simulink model "MiL"  (R2026a)
settings: Solver=FixedStepAuto  StartTime=0  StopTime=2  FixedStep=1e-3  MaxStep=1e-3  EnableMultiTasking=on
values from neighbouring files (symbols this model uses):
  effective_bulkmodulus = 750e6    (= 750000000)    [parameters.m]
  m_load = 58    [parameters.m]
  p_supply = 90e5    (= 9000000)    [parameters.m]
  p_tank = 1.01325e5    (= 101325)    [parameters.m]
undefined symbols (not defined in the file or in its folder): cyl, pipe, valve
libraries: slpidlib x1
settings Model: Creator=ranta34  LastModifiedBy=Lenovo Yoga
settings DataIOCC: SignalLoggingSaveFormat=ModelDataLogs  TimeSaveName=t_sim  Refine=3
settings OptimizationCC: InitFltsAndDblsToZero=on
settings DebuggingCC: SaveWithParameterizedLinksMsg=none  UnderspecifiedInitializationDetection=Classic  SignalResolutionControl=TryResolveAllWithWarning  MinStepSizeMsg=error  MultiTaskDSMMsg=warning  MultiTaskCondExecSysMsg=none
settings HardwareCC: ProdHWDeviceType=32-bit Generic
settings GRTTargetCC: TargetFcnLib=ansi_tfl_tmw.mat  CombineOutputUpdateFcns=off  GRTInterface=on

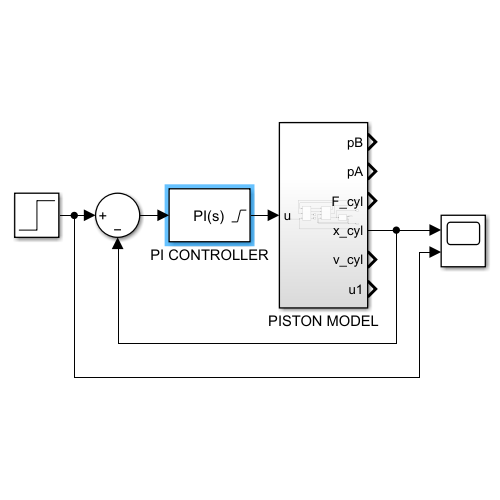
[thumbnail: Simulink's stored preview of the top-level diagram]
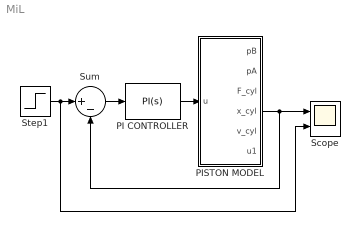
== system MiL ==
  PI CONTROLLER : slpidlib/PID Controller  Controller=PI  Form=Parallel  TimeDomain=Continuous-time  UseExternalTs=off  SampleTime=-1  IntegratorMethod=Forward Euler  FilterMethod=Forward Euler  ControllerParametersSource=internal  P=60  I=1  UseKiTs=off  D=0  UseExternalDerivativeSource=off  N=100  UseFilter=on  TunerSelectOption=Transfer Function Based (PID Tuner App)  InitialConditionSource=internal  InitialConditionForIntegrator=0  InitialConditionForFilter=0  DifferentiatorICPrevScaledInput=0  ExternalReset=none  TrackingMode=off  Kt=1  LimitOutput=on  SatLimitsSource=internal  UpperSaturationLimit=1  LowerSaturationLimit=-1  LinearizeAsGain=on  AntiWindupMode=clamping  Kb=1  LimitIntegrator=off  UpperIntegratorSaturationLimit=inf  LowerIntegratorSaturationLimit=-inf  POutMin=[]  POutMax=[]  IOutMin=[]  IOutMax=[]  DOutMin=[]  DOutMax=[]  NOutMin=[]  NOutMax=[]  SumOutMin=[]  SumOutMax=[]  SaturationOutMin=[]  SaturationOutMax=[]  PParamMin=[]  PParamMax=[]  IParamMin=[]  IParamMax=[]  DParamMin=[]  DParamMax=[]  NParamMin=[]  NParamMax=[]  KbParamMin=[]  KbParamMax=[]  KtParamMin=[]  KtParamMax=[]  KbOutMin=[]  KbOutMax=[]  KtOutMin=[]  KtOutMax=[]  IntegratorOutMin=[]  IntegratorOutMax=[]  FilterOutMin=[]  FilterOutMax=[]  SumI1OutMin=[]  SumI1OutMax=[]  SumI2OutMin=[]  SumI2OutMax=[]  SumI3OutMin=[]  SumI3OutMax=[]  SumI4OutMin=[]  SumI4OutMax=[]  SumDOutMin=[]  SumDOutMax=[]  DifferentiatorOutMin=[]  DifferentiatorOutMax=[]  FilterDiffOutCoefMin=[]  FilterDiffOutCoefMax=[]  ReciprocalOutMin=[]  ReciprocalOutMax=[]  SumDenOutMin=[]  SumDenOutMax=[]  SumNumOutMin=[]  SumNumOutMax=[]  DivideOutMin=[]  DivideOutMax=[]  UdiffTsProdOutMin=[]  UdiffTsProdOutMax=[]  NTsProdOutMin=[]  NTsProdOutMax=[]  UintegralTsProdOutMin=[]  UintegralTsProdOutMax=[]  UngainTsProdOutMin=[]  UngainTsProdOutMax=[]  ClampingZeroOutDataTypeStr=Inherit: Inherit via back propagation  ClampingZeroOutMin=[]  ClampingZeroOutMax=[]  FilterDenConstantOutDataTypeStr=Inherit: Inherit via back propagation  FilterDenConstantOutMin=[]  FilterDenConstantOutMax=[]  PCopyOutDataTypeStr=Inherit: Inherit via back propagation  PCopyOutMin=[]  PCopyOutMax=[]  NCopyOutDataTypeStr=Inherit: Inherit via back propagation  NCopyOutMin=[]  NCopyOutMax=[]  IntegratorContinuousStateAttributes=''  IntegratorStateMustResolveToSignalObject=off  IntegratorRTWStateStorageClass=Auto  FilterContinuousStateAttributes=''  FilterStateMustResolveToSignalObject=off  FilterRTWStateStorageClass=Auto  ParallelPVariant=InternalParameters  IdealPVariant=Disabled  IVariant=InternalParameters  DVariant=Disabled  IntegratorVariant=Continuous  SatVariant=Enabled  AWVariant=ContClampingParallel  PCopyVariant=Disabled  TRVariant=Disabled  FdbkBlocksVariant=Forward  IdealPFdbkVariant=Disabled  SatFdbkVariant=Disabled  DerivativeFilterVariant=Disabled  NVariant=Disabled  NCopyVariant=Disabled_SignalSpec  FilterICVariant=Disabled  IntegratorICVariant=InternalICs  ExternalResetVariant=Disabled  TRSumVariant=Passthrough  SumFdbkVariant=Disabled  SumVariant=Sum_PI  TsampFilterVariant=InternalTs  TsampNgainVariant=Passthrough  TsampIntegralVariant=Disabled_SignalSpec  ExternalSaturationOutDataTypeStr=Inherit: Same as second input  DerivativeSourceVariant=Disabled  PreIntVariant=InternalPreInt
  PISTON MODEL : Subsystem
  Scope : Scope  NumInputPorts=2
      settings: ActiveDisplayYMinimum=-0.44593920723278446  ActiveDisplayYMaximum=1.0292768833436203
  Step1 : Step  Time=0.5  FinalValue=0.40  SampleTime=0
  Sum : Sum  Inputs=|+-
  wires:
  Sum/1 -> PI CONTROLLER/1
  Step1/1 -> Scope/2, Sum/1
  PISTON MODEL/4(x_cyl) -> Scope/1, Sum/2
  PI CONTROLLER/1 -> PISTON MODEL/1(u)

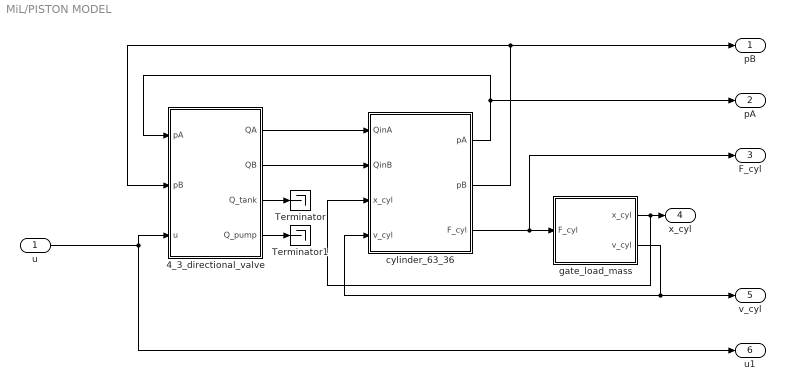
== system MiL/PISTON MODEL ==
  u : Inport
  4_3_directional_valve : Subsystem
  Terminator : Terminator
  Terminator1 : Terminator
  cylinder_63_36 : Subsystem
  gate_load_mass : Subsystem
  pB : Outport
  pA : Outport  Port=2
  F_cyl : Outport  Port=3
  x_cyl : Outport  Port=4
  v_cyl : Outport  Port=5
  u1 : Outport  Port=6
  wires:
  u/1 -> u1/1, 4_3_directional_valve/3(u)
  cylinder_63_36/1(pA) -> pA/1, 4_3_directional_valve/1(pA)
  cylinder_63_36/2(pB) -> pB/1, 4_3_directional_valve/2(pB)
  4_3_directional_valve/1(QA) -> cylinder_63_36/1(QinA)
  4_3_directional_valve/2(QB) -> cylinder_63_36/2(QinB)
  4_3_directional_valve/4(Q_pump) -> Terminator1/1
  4_3_directional_valve/3("Q_tank ") -> Terminator/1
  cylinder_63_36/3(F_cyl) -> F_cyl/1, gate_load_mass/1(F_cyl)
  gate_load_mass/2(v_cyl) -> v_cyl/1, cylinder_63_36/4(v_cyl)
  gate_load_mass/1(x_cyl) -> cylinder_63_36/3(x_cyl), x_cyl/1

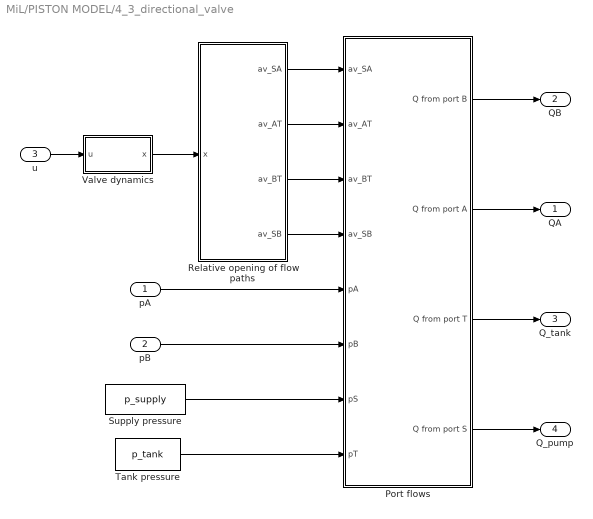
== system MiL/PISTON MODEL/4_3_directional_valve ==
  pA : Inport
  pB : Inport  Port=2
  u : Inport  Port=3
  Port flows : Subsystem
  Relative opening of flow paths : Subsystem
  Supply pressure : Constant  Value=p_supply
  Tank pressure : Constant  Value=p_tank
  Valve dynamics : Subsystem
  QA : Outport  VectorParamsAs1DForOutWhenUnconnected=off
  QB : Outport  Port=2  VectorParamsAs1DForOutWhenUnconnected=off
  "Q_tank " : Outport  Port=3  VectorParamsAs1DForOutWhenUnconnected=off
  Q_pump : Outport  Port=4  VectorParamsAs1DForOutWhenUnconnected=off
  wires:
  pA/1 -> Port flows/5(pA)
  pB/1 -> Port flows/6(pB)
  Valve dynamics/1(x) -> Relative opening of flow paths/1(x)
  Port flows/3(Q from port T) -> "Q_tank "/1
  Port flows/4(Q from port S) -> Q_pump/1
  Relative opening of flow paths/1(av_SA) -> Port flows/1(av_SA)
  Relative opening of flow paths/2(av_AT) -> Port flows/2(av_AT)
  Relative opening of flow paths/4(av_SB) -> Port flows/4(av_SB)
  u/1 -> Valve dynamics/1(u)
  Port flows/2(Q from port A) -> QA/1
  Port flows/1(Q from port B) -> QB/1
  Supply pressure/1 -> Port flows/7(pS)
  Tank pressure/1 -> Port flows/8(pT)
  Relative opening of flow paths/3(av_BT) -> Port flows/3(av_BT)

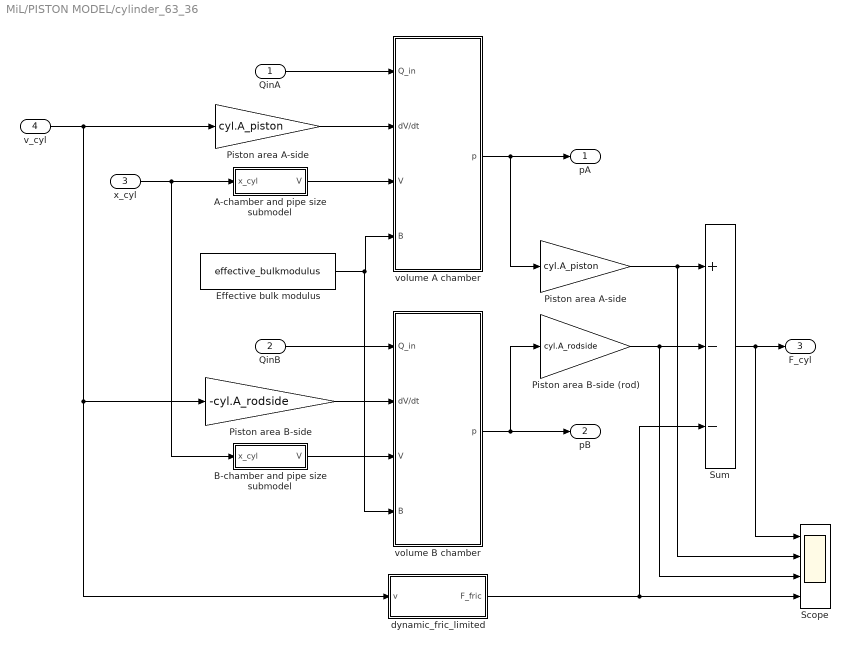
== system MiL/PISTON MODEL/cylinder_63_36 ==
  QinA : Inport
  QinB : Inport  Port=2
  x_cyl : Inport  Port=3
  v_cyl : Inport  Port=4
  A-chamber and pipe size submodel : Subsystem
  B-chamber and pipe size submodel : Subsystem
  Effective bulk modulus : Constant  Value=effective_bulkmodulus
  Piston area A-side : Gain  Gain=cyl.A_piston
  Piston area B-side (rod) : Gain  Gain=cyl.A_rodside
  Piston area A-side : Gain  Gain=cyl.A_piston
  Piston area B-side : Gain  Gain=-cyl.A_rodside
  Scope : Scope  NumInputPorts=4
      settings: ActiveDisplayYMinimum=-3356.48237  ActiveDisplayYMaximum=15799.75819
  Sum : Sum  Inputs=+--
  dynamic_fric_limited : Subsystem
  volume A chamber : Subsystem
  volume B chamber : Subsystem
  pA : Outport  VectorParamsAs1DForOutWhenUnconnected=off
  pB : Outport  Port=2  VectorParamsAs1DForOutWhenUnconnected=off
  F_cyl : Outport  Port=3  VectorParamsAs1DForOutWhenUnconnected=off
  wires:
  Piston area A-side/1 -> Scope/2, Sum/1
  volume A chamber/1(p) -> pA/1, Piston area A-side/1
  x_cyl/1 -> B-chamber and pipe size submodel/1(x_cyl), A-chamber and pipe size submodel/1(x_cyl)
  v_cyl/1 -> dynamic_fric_limited/1(v), Piston area B-side/1, Piston area A-side/1
  Piston area A-side/1 -> volume A chamber/2(" dV/dt")
  Effective bulk modulus/1 -> volume B chamber/4(" B"), volume A chamber/4(" B")
  Sum/1 -> Scope/1, F_cyl/1
  QinA/1 -> volume A chamber/1(Q_in)
  volume B chamber/1(p) -> pB/1, Piston area B-side (rod)/1
  Piston area B-side (rod)/1 -> Scope/3, Sum/2
  A-chamber and pipe size submodel/1(V) -> volume A chamber/3(" V")
  QinB/1 -> volume B chamber/1(Q_in)
  B-chamber and pipe size submodel/1(V) -> volume B chamber/3(" V")
  Piston area B-side/1 -> volume B chamber/2(" dV/dt")
  dynamic_fric_limited/1(F_fric) -> Sum/3, Scope/4

== system MiL/PISTON MODEL/gate_load_mass ==
  F_cyl : Inport
  Add : Sum
  Gain : Gain  Gain=1/m_load
  Integrator : Integrator
  Integrator1 : Integrator  InitialCondition=cyl.x_init
  load_fric : Subsystem
  x_cyl : Outport  VectorParamsAs1DForOutWhenUnconnected=off
  v_cyl : Outport  Port=2  VectorParamsAs1DForOutWhenUnconnected=off
  wires:
  Add/1 -> Gain/1
  Gain/1 -> Integrator/1  "accel"
  Integrator/1 -> load_fric/1(v), v_cyl/1, Integrator1/1  "velocity"
  Integrator1/1 -> x_cyl/1  "position"
  F_cyl/1 -> Add/1
  load_fric/1(F_fric_load) -> Add/2

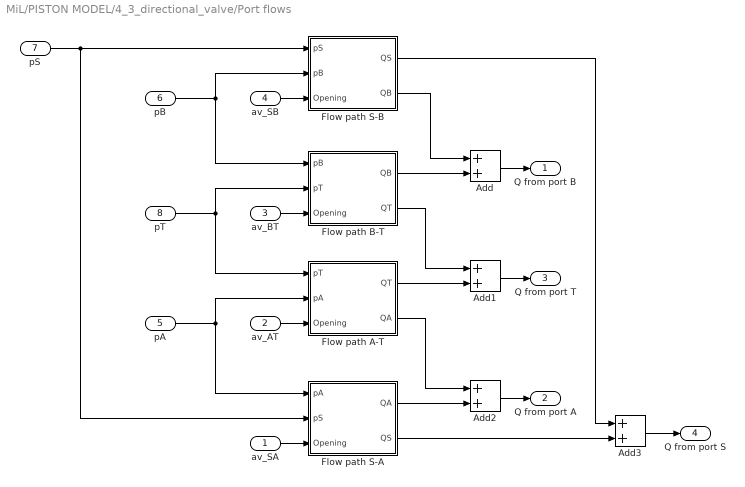
== system MiL/PISTON MODEL/4_3_directional_valve/Port flows ==
  av_SA : Inport
  av_AT : Inport  Port=2
  av_BT : Inport  Port=3
  av_SB : Inport  Port=4
  pA : Inport  Port=5
  pB : Inport  Port=6
  pS : Inport  Port=7
  pT : Inport  Port=8
  Add{,1..3} (4 alike) : Sum
  Flow path A-T : Subsystem  mask(Hydraulic){DPN=valve.dpN, QN=valve.QN, ptr=valve.ptr}
      mask prompts: DPN "Nominal Pressure Difference [Pa] :"; QN "Flow at nominal pressure difference and maximum opening [m^3/s] :"; ptr "Transition pressure [Pa] :"
      mask help:
      | Implements numerically robust turbulent flow equation. Polynomial flow equation is
      | used when abs(dp) is smaller than transition pressure.
      | [Source: Ellman, A. & Piche, R. 1996.
      | A Modified Orifice Flow Formula for Numerical Simulation of Fluid Power Systems.
      | Fluid Power Systems and Technology, ASME]
      mask init:
      | K = QN/(sqrt(DPN));
  Flow path B-T : Subsystem  mask(Hydraulic){DPN=valve.dpN, QN=valve.QN, ptr=valve.ptr}
      mask prompts: DPN "Nominal Pressure Difference [Pa] :"; QN "Flow at nominal pressure difference and maximum opening [m^3/s] :"; ptr "Transition pressure [Pa] :"
      mask help:
      | Implements numerically robust turbulent flow equation. Polynomial flow equation is
      | used when abs(dp) is smaller than transition pressure.
      | [Source: Ellman, A. & Piche, R. 1996.
      | A Modified Orifice Flow Formula for Numerical Simulation of Fluid Power Systems.
      | Fluid Power Systems and Technology, ASME]
      mask init:
      | K = QN/(sqrt(DPN));
  Flow path S-A : Subsystem  mask(Hydraulic){DPN=valve.dpN, QN=valve.QN, ptr=valve.ptr}
      mask prompts: DPN "Nominal Pressure Difference [Pa] :"; QN "Flow at nominal pressure difference and maximum opening [m^3/s] :"; ptr "Transition pressure [Pa] :"
      mask help:
      | Implements numerically robust turbulent flow equation. Polynomial flow equation is
      | used when abs(dp) is smaller than transition pressure.
      | [Source: Ellman, A. & Piche, R. 1996.
      | A Modified Orifice Flow Formula for Numerical Simulation of Fluid Power Systems.
      | Fluid Power Systems and Technology, ASME]
      mask init:
      | K = QN/(sqrt(DPN));
  Flow path S-B : Subsystem  mask(Hydraulic){DPN=valve.dpN, QN=valve.QN, ptr=valve.ptr}
      mask prompts: DPN "Nominal Pressure Difference [Pa] :"; QN "Flow at nominal pressure difference and maximum opening [m^3/s] :"; ptr "Transition pressure [Pa] :"
      mask help:
      | Implements numerically robust turbulent flow equation. Polynomial flow equation is
      | used when abs(dp) is smaller than transition pressure.
      | [Source: Ellman, A. & Piche, R. 1996.
      | A Modified Orifice Flow Formula for Numerical Simulation of Fluid Power Systems.
      | Fluid Power Systems and Technology, ASME]
      mask init:
      | K = QN/(sqrt(DPN));
  Q from port B : Outport  VectorParamsAs1DForOutWhenUnconnected=off
  Q from port A : Outport  Port=2  VectorParamsAs1DForOutWhenUnconnected=off
  Q from port T : Outport  Port=3  VectorParamsAs1DForOutWhenUnconnected=off
  Q from port S : Outport  Port=4  VectorParamsAs1DForOutWhenUnconnected=off
  wires:
  av_SA/1 -> Flow path S-A/3(Opening)
  av_AT/1 -> Flow path A-T/3(Opening)
  av_BT/1 -> Flow path B-T/3(Opening)
  pA/1 -> Flow path A-T/2(pA), Flow path S-A/1(pA)
  pB/1 -> Flow path B-T/1(pB), Flow path S-B/2(pB)
  pS/1 -> Flow path S-B/1(pS), Flow path S-A/2(pS)
  pT/1 -> Flow path A-T/1(pT), Flow path B-T/2(pT)
  Add/1 -> Q from port B/1
  Add1/1 -> Q from port T/1
  Add2/1 -> Q from port A/1
  Add3/1 -> Q from port S/1
  Flow path S-B/1(QS) -> Add3/1
  Flow path S-A/2(QS) -> Add3/2
  Flow path S-A/1(QA) -> Add2/2
  Flow path A-T/2(QA) -> Add2/1
  Flow path A-T/1(QT) -> Add1/2
  Flow path B-T/2(QT) -> Add1/1
  Flow path B-T/1(QB) -> Add/2
  Flow path S-B/2(QB) -> Add/1
  av_SB/1 -> Flow path S-B/3(Opening)

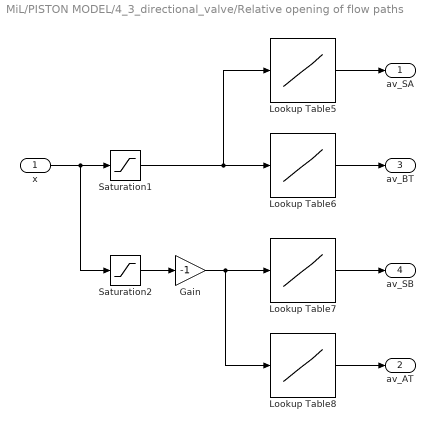
== system MiL/PISTON MODEL/4_3_directional_valve/Relative opening of flow paths ==
  x : Inport
  Gain : Gain  Gain=-1
  Lookup Table5 : Lookup  InputValues=[0.01 0.05 0.1 0.2 0.3 0.4 1]  Table=[0.01 0.039 0.078 0.16 0.23 0.31 0.78]  SaturateOnIntegerOverflow=off
  Lookup Table6 : Lookup  InputValues=[0.01 0.05 0.1 0.2 0.3 0.4 1]  Table=[0.01 0.036 0.072 0.14 0.22 0.29 0.72]  SaturateOnIntegerOverflow=off
  Lookup Table7 : Lookup  InputValues=[0.01 0.05 0.1 0.2 0.3 0.4 1]  Table=[0.01 0.039 0.077 0.15 0.23 0.31 0.77]  SaturateOnIntegerOverflow=off
  Lookup Table8 : Lookup  InputValues=[0.01 0.05 0.1 0.2 0.3 0.4 1]  Table=[0.01 0.035 0.070 0.14 0.21 0.28 0.70]  SaturateOnIntegerOverflow=off
  Saturation1 : Saturate  UpperLimit=1  LowerLimit=0
  Saturation2 : Saturate  UpperLimit=0  LowerLimit=-1
  av_SA : Outport  VectorParamsAs1DForOutWhenUnconnected=off
  av_AT : Outport  Port=2  VectorParamsAs1DForOutWhenUnconnected=off
  av_BT : Outport  Port=3  VectorParamsAs1DForOutWhenUnconnected=off
  av_SB : Outport  Port=4  VectorParamsAs1DForOutWhenUnconnected=off
  wires:
  x/1 -> Saturation2/1, Saturation1/1
  Saturation2/1 -> Gain/1
  Lookup Table8/1 -> av_AT/1
  Lookup Table7/1 -> av_SB/1
  Lookup Table6/1 -> av_BT/1
  Lookup Table5/1 -> av_SA/1
  Saturation1/1 -> Lookup Table5/1, Lookup Table6/1
  Gain/1 -> Lookup Table8/1, Lookup Table7/1

== system MiL/PISTON MODEL/4_3_directional_valve/Valve dynamics ==
  u : Inport
  Rate Limiter : RateLimiter  RisingSlewLimit=valve.ratelimit  FallingSlewLimit=-valve.ratelimit  SampleTimeMode=inherited
  Saturation limits [-1,1] : Saturate  UpperLimit=1  LowerLimit=-1
  Saturation limits [-1,1]2 : Saturate  UpperLimit=1  LowerLimit=-1
  Transfer Fcn1 : TransferFcn  Denominator=[valve.tau 1]
  Transport Delay of the valve : TransportDelay  DelayTime=valve.delay
  x : Outport  VectorParamsAs1DForOutWhenUnconnected=off
  wires:
  Saturation limits [-1,1]/1 -> Transport Delay of the valve/1
  Transport Delay of the valve/1 -> Rate Limiter/1
  Rate Limiter/1 -> Transfer Fcn1/1
  u/1 -> Saturation limits [-1,1]/1
  Transfer Fcn1/1 -> Saturation limits [-1,1]2/1
  Saturation limits [-1,1]2/1 -> x/1

== system MiL/PISTON MODEL/cylinder_63_36/A-chamber and pipe size submodel ==
  x_cyl : Inport
  A : Gain  Gain=pipe.area
  A chamber dead volume : Constant  Value=cyl.V0A
  Add : Sum  Inputs=+++
  Gain : Gain  Gain=cyl.A_piston
  Lenght : Constant  Value=pipe.lenght
  V : Outport  VectorParamsAs1DForOutWhenUnconnected=off
  wires:
  A/1 -> Add/3
  Lenght/1 -> A/1
  A chamber dead volume/1 -> Add/2
  Gain/1 -> Add/1
  x_cyl/1 -> Gain/1
  Add/1 -> V/1

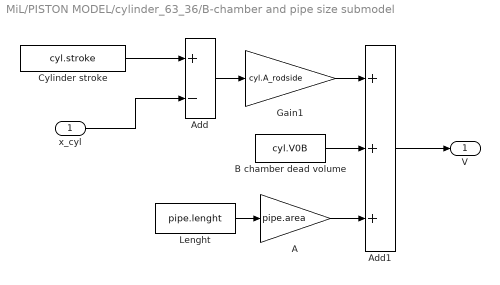
== system MiL/PISTON MODEL/cylinder_63_36/B-chamber and pipe size submodel ==
  x_cyl : Inport
  A : Gain  Gain=pipe.area
  Add : Sum  Inputs=+-
  Add1 : Sum  Inputs=+++
  B chamber dead volume : Constant  Value=cyl.V0B
  Cylinder stroke : Constant  Value=cyl.stroke
  Gain1 : Gain  Gain=cyl.A_rodside
  Lenght : Constant  Value=pipe.lenght
  V : Outport  VectorParamsAs1DForOutWhenUnconnected=off
  wires:
  A/1 -> Add1/3
  Lenght/1 -> A/1
  Cylinder stroke/1 -> Add/1
  Gain1/1 -> Add1/1
  Add/1 -> Gain1/1
  x_cyl/1 -> Add/2
  B chamber dead volume/1 -> Add1/2
  Add1/1 -> V/1

== system MiL/PISTON MODEL/cylinder_63_36/dynamic_fric_limited ==
  v : Inport
  Abs : Abs  SaturateOnIntegerOverflow=off
  Product : Product
  Sign : Signum
  cyl_fric_up_to_100mm/s : Lookup_n-D  NumberOfTableDimensions=1  BreakpointsForDimension1=|  Table=|  InternalRulePriority=Speed  RndMeth=Simplest
      BreakpointsForDimension1=|
      | [0
      | 5
      | 10
      | 15
      | 20
      | 25
      | 30
      | 35
      | 40
      | 45
      | 50
      | 55
      | 60
      | 65
      | 70
      | 75
      | 80
      | 85
      | 90
      | 95
      | 100]./1e3;
      Table=|
      | [0
      | 242
      | 550
      | 838
      | 996
      | 972
      | 850
      | 757
      | 728
      | 733
      | 744
      | 753
      | 759
      | 765
      | 770
      | 775
      | 780
      | 785
      | 790
      | 795
      | 800];
  F_fric : Outport  VectorParamsAs1DForOutWhenUnconnected=off
  wires:
  Abs/1 -> cyl_fric_up_to_100mm/s/1
  v/1 -> Sign/1, Abs/1
  cyl_fric_up_to_100mm/s/1 -> Product/1
  Sign/1 -> Product/2
  Product/1 -> F_fric/1

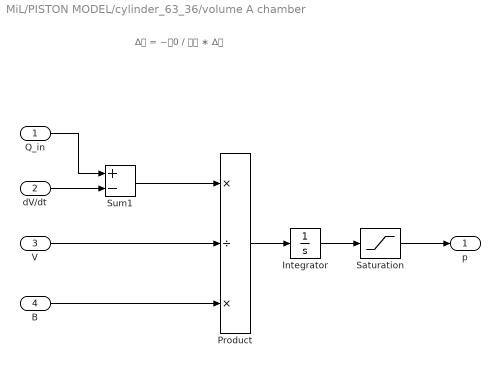
== system MiL/PISTON MODEL/cylinder_63_36/volume A chamber ==
  note: ∆𝑉 = −𝑉0 / 𝐵𝑛 ∗ ∆𝑝
  Q_in : Inport
  " dV/dt" : Inport  Port=2
  " V" : Inport  Port=3
  " B" : Inport  Port=4
  Integrator : Integrator  InitialCondition=cyl.p0A  AbsoluteTolerance=10
  Product : Product  Inputs=*/*  InputSameDT=on  SaturateOnIntegerOverflow=on  OutDataTypeStr=Inherit: Same as first input
  Saturation : Saturate  UpperLimit=inf  LowerLimit=-1e5
  Sum1 : Sum  Inputs=+-  InputSameDT=on  SaturateOnIntegerOverflow=on  OutDataTypeStr=Inherit: Same as first input
  p : Outport  VectorParamsAs1DForOutWhenUnconnected=off
  wires:
  Integrator/1 -> Saturation/1
  Product/1 -> Integrator/1
  Sum1/1 -> Product/1
  " B"/1 -> Product/3
  Saturation/1 -> p/1
  Q_in/1 -> Sum1/1
  " V"/1 -> Product/2
  " dV/dt"/1 -> Sum1/2

== system MiL/PISTON MODEL/cylinder_63_36/volume B chamber ==
  Q_in : Inport
  " dV/dt" : Inport  Port=2
  " V" : Inport  Port=3
  " B" : Inport  Port=4
  Integrator : Integrator  InitialCondition=cyl.p0B  AbsoluteTolerance=10
  Product : Product  Inputs=*/*  InputSameDT=on  SaturateOnIntegerOverflow=on  OutDataTypeStr=Inherit: Same as first input
  Saturation : Saturate  UpperLimit=inf  LowerLimit=-1e5
  Sum1 : Sum  Inputs=+-  InputSameDT=on  SaturateOnIntegerOverflow=on  OutDataTypeStr=Inherit: Same as first input
  p : Outport  VectorParamsAs1DForOutWhenUnconnected=off
  wires:
  " dV/dt"/1 -> Sum1/2
  " V"/1 -> Product/2
  Q_in/1 -> Sum1/1
  Saturation/1 -> p/1
  " B"/1 -> Product/3
  Sum1/1 -> Product/1
  Product/1 -> Integrator/1
  Integrator/1 -> Saturation/1

== system MiL/PISTON MODEL/gate_load_mass/load_fric ==
  v : Inport
  Gain1 : Gain  Gain=-1
  Product : Product  Inputs=4
  Sign : Signum
  coeff_fric : Constant  Value=0.7e5
  F_fric_load : Outport  VectorParamsAs1DForOutWhenUnconnected=off
  wires:
  Product/1 -> F_fric_load/1
  Sign/1 -> Gain1/1
  coeff_fric/1 -> Product/4
  Gain1/1 -> Product/1
  v/1 -> Product/2, Product/3, Sign/1

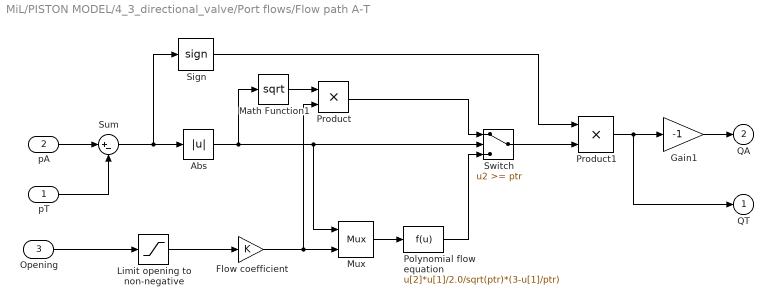
== system MiL/PISTON MODEL/4_3_directional_valve/Port flows/Flow path A-T ==
  pT : Inport
  pA : Inport  Port=2
  Opening : Inport  Port=3
  Abs : Abs  ZeroCross=off
  Flow coefficient : Gain  Gain=K  SaturateOnIntegerOverflow=on  OutDataTypeStr=Inherit: Same as input  ParamDataTypeStr=Inherit: Same as input
  Gain1 : Gain  Gain=-1  SaturateOnIntegerOverflow=on  OutDataTypeStr=Inherit: Same as input  ParamDataTypeStr=Inherit: Same as input
  Limit opening to non-negative : Saturate  UpperLimit=inf  LowerLimit=0
  Math Function1 : Math  Operator=sqrt  SignedPower=on
  Mux : Mux  Inputs=2
  Polynomial flow equation : Fcn  Expr=u[2]*u[1]/2.0/sqrt(ptr)*(3-u[1]/ptr)
  Product : Product  InputSameDT=on  SaturateOnIntegerOverflow=on  OutDataTypeStr=Inherit: Same as first input
  Product1 : Product  InputSameDT=on  SaturateOnIntegerOverflow=on  OutDataTypeStr=Inherit: Same as first input
  Sign : Signum  ZeroCross=off
  Sum : Sum  Inputs=|+-
  Switch : Switch  Threshold=ptr  ZeroCross=off
  QT : Outport  InitialOutput=0  VectorParamsAs1DForOutWhenUnconnected=off
  QA : Outport  Port=2  InitialOutput=0  VectorParamsAs1DForOutWhenUnconnected=off
  wires:
  Opening/1 -> Limit opening to non-negative/1
  Sum/1 -> Abs/1, Sign/1
  Polynomial flow equation/1 -> Switch/3
  Mux/1 -> Polynomial flow equation/1
  Product/1 -> Switch/1
  Math Function1/1 -> Product/1
  Abs/1 -> Mux/1, Switch/2, Math Function1/1
  Limit opening to non-negative/1 -> Flow coefficient/1
  Flow coefficient/1 -> Product/2, Mux/2
  Sign/1 -> Product1/1
  Product1/1 -> Gain1/1, QT/1
  Switch/1 -> Product1/2
  pA/1 -> Sum/1
  pT/1 -> Sum/2
  Gain1/1 -> QA/1

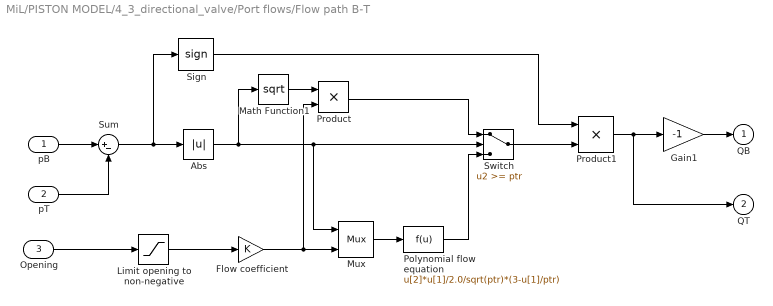
== system MiL/PISTON MODEL/4_3_directional_valve/Port flows/Flow path B-T ==
  pB : Inport
  pT : Inport  Port=2
  Opening : Inport  Port=3
  Abs : Abs  ZeroCross=off
  Flow coefficient : Gain  Gain=K  SaturateOnIntegerOverflow=on  OutDataTypeStr=Inherit: Same as input  ParamDataTypeStr=Inherit: Same as input
  Gain1 : Gain  Gain=-1  SaturateOnIntegerOverflow=on  OutDataTypeStr=Inherit: Same as input  ParamDataTypeStr=Inherit: Same as input
  Limit opening to non-negative : Saturate  UpperLimit=inf  LowerLimit=0
  Math Function1 : Math  Operator=sqrt  SignedPower=on
  Mux : Mux  Inputs=2
  Polynomial flow equation : Fcn  Expr=u[2]*u[1]/2.0/sqrt(ptr)*(3-u[1]/ptr)
  Product : Product  InputSameDT=on  SaturateOnIntegerOverflow=on  OutDataTypeStr=Inherit: Same as first input
  Product1 : Product  InputSameDT=on  SaturateOnIntegerOverflow=on  OutDataTypeStr=Inherit: Same as first input
  Sign : Signum  ZeroCross=off
  Sum : Sum  Inputs=|+-
  Switch : Switch  Threshold=ptr  ZeroCross=off
  QB : Outport  InitialOutput=0  VectorParamsAs1DForOutWhenUnconnected=off
  QT : Outport  Port=2  InitialOutput=0  VectorParamsAs1DForOutWhenUnconnected=off
  wires:
  Gain1/1 -> QB/1
  pT/1 -> Sum/2
  pB/1 -> Sum/1
  Switch/1 -> Product1/2
  Product1/1 -> QT/1, Gain1/1
  Sign/1 -> Product1/1
  Flow coefficient/1 -> Mux/2, Product/2
  Limit opening to non-negative/1 -> Flow coefficient/1
  Abs/1 -> Math Function1/1, Switch/2, Mux/1
  Math Function1/1 -> Product/1
  Product/1 -> Switch/1
  Mux/1 -> Polynomial flow equation/1
  Polynomial flow equation/1 -> Switch/3
  Sum/1 -> Sign/1, Abs/1
  Opening/1 -> Limit opening to non-negative/1

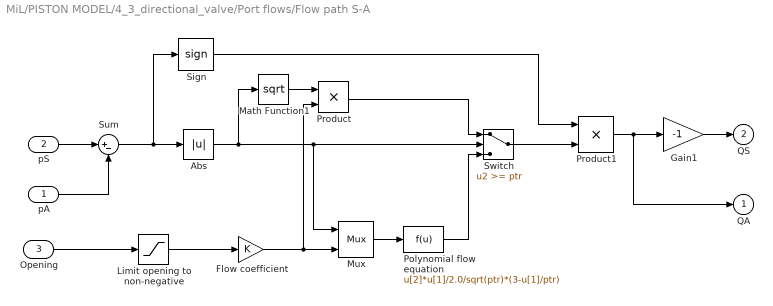
== system MiL/PISTON MODEL/4_3_directional_valve/Port flows/Flow path S-A ==
  pA : Inport
  pS : Inport  Port=2
  Opening : Inport  Port=3
  Abs : Abs  ZeroCross=off
  Flow coefficient : Gain  Gain=K  SaturateOnIntegerOverflow=on  OutDataTypeStr=Inherit: Same as input  ParamDataTypeStr=Inherit: Same as input
  Gain1 : Gain  Gain=-1  SaturateOnIntegerOverflow=on  OutDataTypeStr=Inherit: Same as input  ParamDataTypeStr=Inherit: Same as input
  Limit opening to non-negative : Saturate  UpperLimit=inf  LowerLimit=0
  Math Function1 : Math  Operator=sqrt  SignedPower=on
  Mux : Mux  Inputs=2
  Polynomial flow equation : Fcn  Expr=u[2]*u[1]/2.0/sqrt(ptr)*(3-u[1]/ptr)
  Product : Product  InputSameDT=on  SaturateOnIntegerOverflow=on  OutDataTypeStr=Inherit: Same as first input
  Product1 : Product  InputSameDT=on  SaturateOnIntegerOverflow=on  OutDataTypeStr=Inherit: Same as first input
  Sign : Signum  ZeroCross=off
  Sum : Sum  Inputs=|+-
  Switch : Switch  Threshold=ptr  ZeroCross=off
  QA : Outport  InitialOutput=0  VectorParamsAs1DForOutWhenUnconnected=off
  QS : Outport  Port=2  InitialOutput=0  VectorParamsAs1DForOutWhenUnconnected=off
  wires:
  Opening/1 -> Limit opening to non-negative/1
  Sum/1 -> Abs/1, Sign/1
  Polynomial flow equation/1 -> Switch/3
  Mux/1 -> Polynomial flow equation/1
  Product/1 -> Switch/1
  Math Function1/1 -> Product/1
  Abs/1 -> Mux/1, Switch/2, Math Function1/1
  Limit opening to non-negative/1 -> Flow coefficient/1
  Flow coefficient/1 -> Product/2, Mux/2
  Sign/1 -> Product1/1
  Product1/1 -> Gain1/1, QA/1
  Switch/1 -> Product1/2
  pS/1 -> Sum/1
  pA/1 -> Sum/2
  Gain1/1 -> QS/1

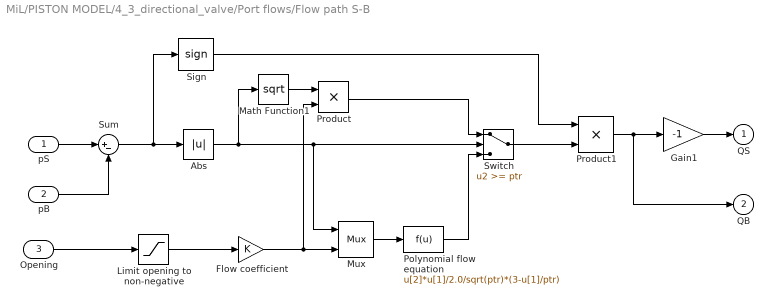
== system MiL/PISTON MODEL/4_3_directional_valve/Port flows/Flow path S-B ==
  pS : Inport
  pB : Inport  Port=2
  Opening : Inport  Port=3
  Abs : Abs  ZeroCross=off
  Flow coefficient : Gain  Gain=K  SaturateOnIntegerOverflow=on  OutDataTypeStr=Inherit: Same as input  ParamDataTypeStr=Inherit: Same as input
  Gain1 : Gain  Gain=-1  SaturateOnIntegerOverflow=on  OutDataTypeStr=Inherit: Same as input  ParamDataTypeStr=Inherit: Same as input
  Limit opening to non-negative : Saturate  UpperLimit=inf  LowerLimit=0
  Math Function1 : Math  Operator=sqrt  SignedPower=on
  Mux : Mux  Inputs=2
  Polynomial flow equation : Fcn  Expr=u[2]*u[1]/2.0/sqrt(ptr)*(3-u[1]/ptr)
  Product : Product  InputSameDT=on  SaturateOnIntegerOverflow=on  OutDataTypeStr=Inherit: Same as first input
  Product1 : Product  InputSameDT=on  SaturateOnIntegerOverflow=on  OutDataTypeStr=Inherit: Same as first input
  Sign : Signum  ZeroCross=off
  Sum : Sum  Inputs=|+-
  Switch : Switch  Threshold=ptr  ZeroCross=off
  QS : Outport  InitialOutput=0  VectorParamsAs1DForOutWhenUnconnected=off
  QB : Outport  Port=2  InitialOutput=0  VectorParamsAs1DForOutWhenUnconnected=off
  wires:
  Gain1/1 -> QS/1
  pB/1 -> Sum/2
  pS/1 -> Sum/1
  Switch/1 -> Product1/2
  Product1/1 -> QB/1, Gain1/1
  Sign/1 -> Product1/1
  Flow coefficient/1 -> Mux/2, Product/2
  Limit opening to non-negative/1 -> Flow coefficient/1
  Abs/1 -> Math Function1/1, Switch/2, Mux/1
  Math Function1/1 -> Product/1
  Product/1 -> Switch/1
  Mux/1 -> Polynomial flow equation/1
  Polynomial flow equation/1 -> Switch/3
  Sum/1 -> Sign/1, Abs/1
  Opening/1 -> Limit opening to non-negative/1
